simulink library "ControlTiming"  (R2026a)
settings: Solver=VariableStepAuto
undefined symbols (not defined in the file): timingCfg
settings Model: Creator=24322  LastModifiedBy=24322

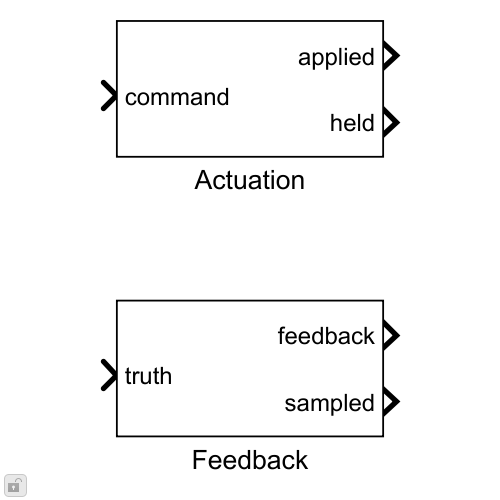
[thumbnail: Simulink's stored preview of the top-level diagram]
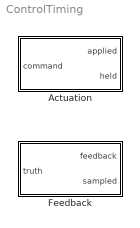
== system ControlTiming ==
  Actuation : Subsystem
  Feedback : Subsystem

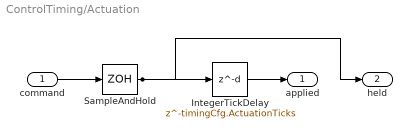
== system ControlTiming/Actuation ==
  command : Inport
  IntegerTickDelay : Delay  DelayLength=timingCfg.ActuationTicks  InitialCondition=0  SampleTime=timingCfg.Ts
  SampleAndHold : ZeroOrderHold  SampleTime=timingCfg.Ts
  applied : Outport
  held : Outport  Port=2
  wires:
  IntegerTickDelay/1 -> applied/1
  SampleAndHold/1 -> IntegerTickDelay/1, held/1
  command/1 -> SampleAndHold/1

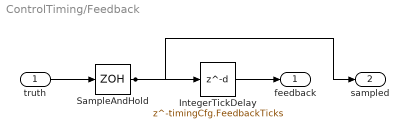
== system ControlTiming/Feedback ==
  truth : Inport
  IntegerTickDelay : Delay  DelayLength=timingCfg.FeedbackTicks  InitialCondition=0  SampleTime=timingCfg.Ts
  SampleAndHold : ZeroOrderHold  SampleTime=timingCfg.Ts
  feedback : Outport
  sampled : Outport  Port=2
  wires:
  IntegerTickDelay/1 -> feedback/1
  SampleAndHold/1 -> IntegerTickDelay/1, sampled/1
  truth/1 -> SampleAndHold/1
